simulink model "LLC_Phase_Shift_R2016a"  (R2016a)
settings: Solver=VariableStepAuto  SolverMode=SingleTasking  StartTime=0.0  StopTime=1  RelTol=1e-3
libraries: powerlib x35, simulink x1
settings Model: Creator=20695  LastModifiedBy=20695
settings DataIOCC: ReturnWorkspaceOutputs=on
settings DebuggingCC: UnconnectedInputMsg=none  UnconnectedOutputMsg=none  UnconnectedLineMsg=none  SFUnexpectedBacktrackingDiag=error  SFNoUnconditionalDefaultTransitionDiag=error
settings ModelReferenceCC: EnableRefExpFcnMdlSchedulingChecks=off
settings SFSimCC: SimUseLocalCustomCode=on
settings RTWCC: Description=Generic Real-Time Target  RTWUseLocalCustomCode=on
settings GRTTargetCC: TargetLangStandard=C99 (ISO)
settings ConfigComp: CovMetricSettings=dwe  CovSaveCumulativeToWorkspaceVar=off  CovSaveSingleToWorkspaceVar=off  CovExternalEMLEnable=on

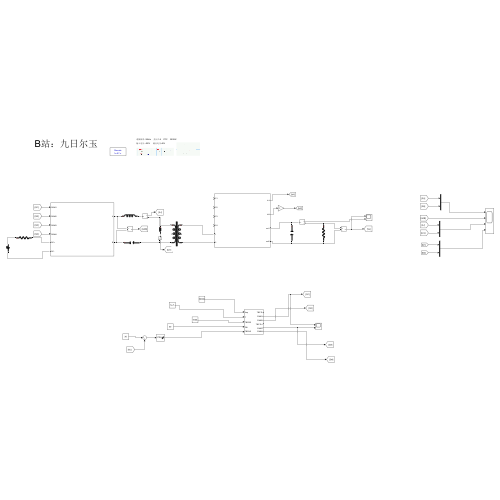
[thumbnail: Simulink's stored preview of the top-level diagram]
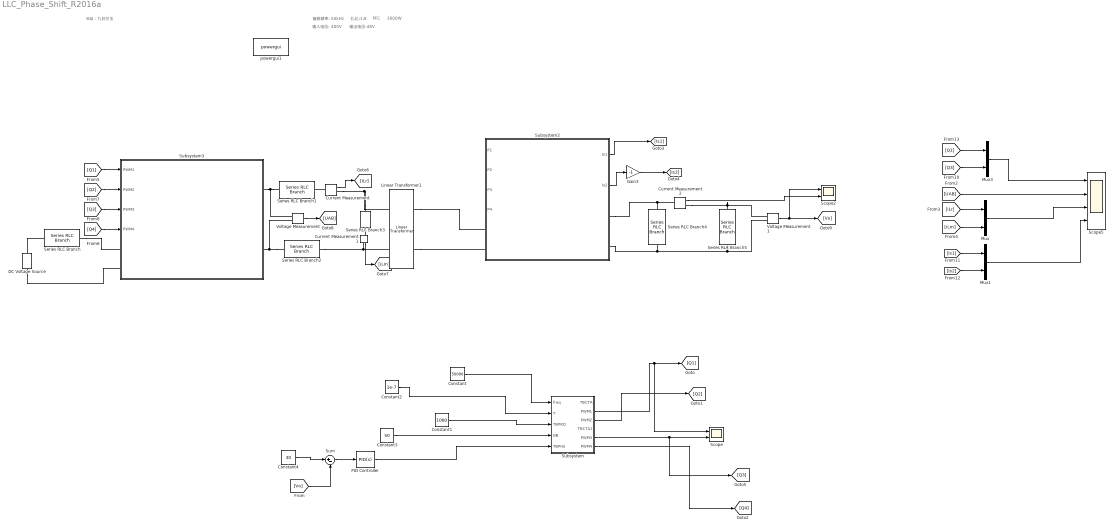
== system LLC_Phase_Shift_R2016a ==
  note: 谐振频率: 50kHz
  note: 输出电压:48V
  note: 3000W
  note: 输入电压: 400V
  note: 扎比:1:8
  note: B站：九日尔玉
  note: PFC
  Constant : Constant  Value=50000
  Constant1 : Constant  Value=1000
  Constant2 : Constant  Value=1e-7
  Constant3 : Constant  Value=50
  Constant4 : Constant  Value=30
  Current Measurement : powerlib/Measurements/Current Measurement  PhasorSimulation=off  OutputType=Complex  PSBequivalent=0
  Current Measurement1 : powerlib/Measurements/Current Measurement  PhasorSimulation=off  OutputType=Complex  PSBequivalent=0
  Current Measurement2 : powerlib/Measurements/Current Measurement  PhasorSimulation=off  OutputType=Complex  PSBequivalent=0
  DC Voltage Source : powerlib/Electrical Sources/DC Voltage Source  Amplitude=400  Measurements=None
  Gain3 : Gain  Gain=-1
  Linear Transformer1 : powerlib/Elements/Linear Transformer  UNITS=SI  NominalPower=[ 3e3 50e3 ]  winding1=[8 0 0]  winding2=[1 0 0]  ThreeWindings=off  winding3=[41.5 1e-4 1e-7]  RmLm=[1e8 0]  Measurements=None  DataType=on
  Mux : Mux  Inputs=2
  Mux1 : Mux  Inputs=2
  Mux3 : Mux  Inputs=2
  PID Controller : simulink/Continuous/PID Controller  Controller=PID  Form=Parallel  TimeDomain=Continuous-time  SampleTime=-1  IntegratorMethod=Forward Euler  ControllerParametersSource=internal  P=100  I=1000  D=0  N=100  UseFilter=on  InitialConditionSource=internal  InitialConditionForIntegrator=0  InitialConditionForFilter=0  DifferentiatorICPrevScaledInput=0  ExternalReset=none  TrackingMode=off  Kt=1  LimitOutput=on  UpperSaturationLimit=1000  LowerSaturationLimit=0  LinearizeAsGain=on  AntiWindupMode=none  Kb=1  POutMin=[]  POutMax=[]  IOutMin=[]  IOutMax=[]  DOutMin=[]  DOutMax=[]  NOutMin=[]  NOutMax=[]  SumOutMin=[]  SumOutMax=[]  SaturationOutMin=[]  SaturationOutMax=[]  PParamMin=[]  PParamMax=[]  IParamMin=[]  IParamMax=[]  DParamMin=[]  DParamMax=[]  NParamMin=[]  NParamMax=[]  KbParamMin=[]  KbParamMax=[]  KtParamMin=[]  KtParamMax=[]  KbOutMin=[]  KbOutMax=[]  KtOutMin=[]  KtOutMax=[]  IntegratorOutMin=[]  IntegratorOutMax=[]  FilterOutMin=[]  FilterOutMax=[]  SumI1OutMin=[]  SumI1OutMax=[]  SumI2OutMin=[]  SumI2OutMax=[]  SumI3OutMin=[]  SumI3OutMax=[]  SumDOutMin=[]  SumDOutMax=[]  DifferentiatorOutMin=[]  DifferentiatorOutMax=[]  IntegratorContinuousStateAttributes=''  IntegratorStateMustResolveToSignalObject=off  IntegratorRTWStateStorageClass=Auto  FilterContinuousStateAttributes=''  FilterStateMustResolveToSignalObject=off  FilterRTWStateStorageClass=Auto
  Scope : Scope  NumInputPorts=2
  Scope2 : Scope  NumInputPorts=2
  Scope5 : Scope  NumInputPorts=4
  Series RLC Branch : powerlib/Elements/Series RLC Branch  LConnTagsString=__new0  RConnTagsString=__new0  BranchType=R  Resistance=0.0001  Inductance=1e-3  SetiL0=off  InitialCurrent=0  Capacitance=1e-6  Setx0=off  InitialVoltage=0  Measurements=None
  Series RLC Branch1 : powerlib/Elements/Series RLC Branch  LConnTagsString=__new0  RConnTagsString=__new0  BranchType=L  Resistance=0.0001  Inductance=0.078e-3  SetiL0=off  InitialCurrent=0  Capacitance=1e-6  Setx0=off  InitialVoltage=0  Measurements=None
  Series RLC Branch2 : powerlib/Elements/Series RLC Branch  LConnTagsString=__new0  RConnTagsString=__new0  BranchType=C  Resistance=0.0001  Inductance=1e-3  SetiL0=off  InitialCurrent=0  Capacitance=130.508e-9  Setx0=off  InitialVoltage=0  Measurements=None
  Series RLC Branch3 : powerlib/Elements/Series RLC Branch  LConnTagsString=__new0  RConnTagsString=__new0  BranchType=L  Resistance=0.0001  Inductance=0.233e-3  SetiL0=off  InitialCurrent=0  Capacitance=1e-6  Setx0=off  InitialVoltage=0  Measurements=None
  Series RLC Branch4 : powerlib/Elements/Series RLC Branch  LConnTagsString=__new0  RConnTagsString=__new0  BranchType=C  Resistance=1  Inductance=1e-3  SetiL0=off  InitialCurrent=0  Capacitance=2e-3  Setx0=on  InitialVoltage=0  Measurements=None
  Series RLC Branch5 : powerlib/Elements/Series RLC Branch  LConnTagsString=__new0  RConnTagsString=__new0  BranchType=R  Resistance=1  Inductance=1e-3  SetiL0=off  InitialCurrent=0  Capacitance=2e-3  Setx0=off  InitialVoltage=0  Measurements=None
  Subsystem : Subsystem
  Subsystem2 : Subsystem  mask{C=0}
  Subsystem3 : Subsystem  mask{C=330e-12}
      mask prompts: C "寄生电容大小"
  Sum : Sum  Inputs=|+-
  Voltage Measurement : powerlib/Measurements/Voltage Measurement  PhasorSimulation=off  OutputType=Complex  PSBequivalent=0
  Voltage Measurement1 : powerlib/Measurements/Voltage Measurement  PhasorSimulation=off  OutputType=Complex  PSBequivalent=0
  powergui1 : powerlib/powergui  Priority=1  SimulationMode=Discrete  SampleTime=1e-7  frequency=60  Iterations=50  frequencyindice=0  Pbase=100e6  ErrMax=1e-4  UnitsV=kV  UnitsW=MW  buscounter=0  FunctionMessages=off  echomessages=off  EnableUseOfTLC=off  CurrentSourceSwitches=off  DisableSnubberDevices=off  DisableRonSwitches=off  DisableVfSwitches=off  DisplayEquations=off  AutomaticDiscreteSolvers=off  SolverType=Tustin/Backward Euler (TBE)  Interpol=off  ExternalGateDelay=off  methode=off  Ts=100  x0status=blocks  SPID=on  SwTol=0  HookPort=off  NonlinearTolerance=1e-4  nMaxIteration=100  ContinueOnMaxIteration=off  RestoreLinks=warning  ResistiveCurrentMeasurement=off  Frange=[0:2:500]  Ylog=off  Xlog=on  ShowGrid=off  save=off  variable=ZData  structure=0  ZoomFFT=off  StartTime=0.0  cycles=1  DisplayStyle=1  fundamental=60  FreqAxis=off  MaxFrequency=1000  frequencyindicesteady=1  RmsSteady=1  display=off
  wires:
  [Q4] -> Subsystem3/4(PWM4)
  [Q2] -> Subsystem3/2(PWM2)
  [Q3] -> Subsystem3/3(PWM3)
  Subsystem2/1(Is1) -> [Is1]
  Current Measurement2/1 -> Scope2/2
  Subsystem2/2(Is2) -> Gain3/1
  Voltage Measurement/1 -> [UAB]
  Voltage Measurement1/1 -> [Vo], Scope2/1
  Gain3/1 -> [Is2]
  [Q1] -> Subsystem3/1(PWM1)
  [UAB] -> Scope5/2
  Mux3/1 -> Scope5/1
  [iLm] -> Mux/2
  Current Measurement/1 -> [iLr]
  [Q3] -> Mux3/2
  Mux/1 -> Scope5/3
  [Q1] -> Mux3/1
  [Is2] -> Mux1/2
  Current Measurement1/1 -> [iLm]
  Mux1/1 -> Scope5/4
  [iLr] -> Mux/1
  [Is1] -> Mux1/1
  Subsystem/2(PWM1) -> Scope/1, [Q1]
  Subsystem/5(PWM3) -> [Q3], Scope/2
  Constant/1 -> Subsystem/1(freq)
  Constant2/1 -> Subsystem/2(T)
  Constant1/1 -> Subsystem/3(TBPRD)
  Constant3/1 -> Subsystem/4(DB)
  PID Controller/1 -> Subsystem/5(TBPHS)
  Subsystem/3(PWM2) -> [Q2]
  Subsystem/6(PWM4) -> [Q4]
  [Vo] -> Sum/2
  Constant4/1 -> Sum/1
  Sum/1 -> PID Controller/1
  connections:
  Series RLC Branch2/LConn1 -- Subsystem3/RConn2 -- Voltage Measurement/LConn2
  Series RLC Branch4/LConn1 -- Subsystem2/RConn1 -- Current Measurement2/LConn1
  Series RLC Branch4/RConn1 -- Subsystem2/RConn2 -- Voltage Measurement1/LConn2 -- Series RLC Branch5/RConn1
  Series RLC Branch3/LConn1 -- Current Measurement/RConn1 -- Linear Transformer1/LConn1
  Series RLC Branch1/LConn1 -- Subsystem3/RConn1 -- Voltage Measurement/LConn1
  Series RLC Branch5/LConn1 -- Current Measurement2/RConn1 -- Voltage Measurement1/LConn1
  Current Measurement1/RConn1 -- Series RLC Branch2/RConn1 -- Linear Transformer1/LConn2
  Linear Transformer1/RConn1 -- Subsystem2/LConn1
  DC Voltage Source/RConn1 -- Series RLC Branch/LConn1
  Current Measurement1/LConn1 -- Series RLC Branch3/RConn1
  Current Measurement/LConn1 -- Series RLC Branch1/RConn1
  Linear Transformer1/RConn2 -- Subsystem2/LConn2
  Series RLC Branch/RConn1 -- Subsystem3/LConn1
  DC Voltage Source/LConn1 -- Subsystem3/LConn2

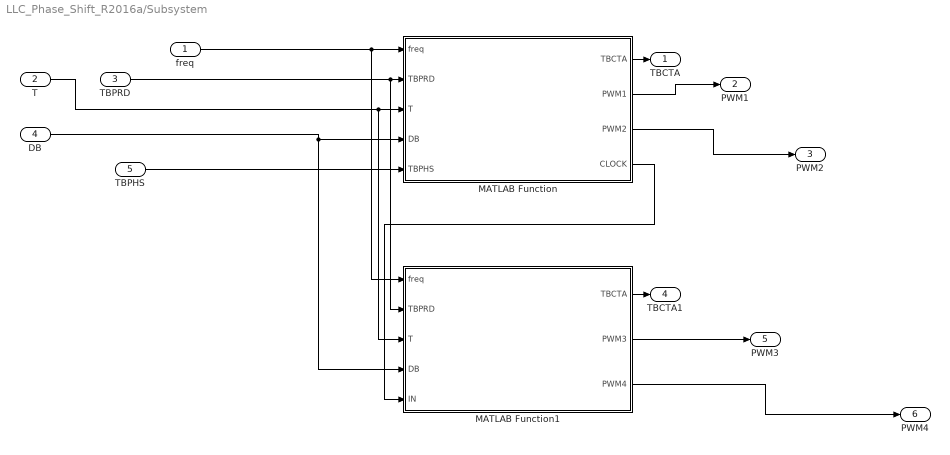
== system LLC_Phase_Shift_R2016a/Subsystem ==
  freq : Inport
  T : Inport  Port=2
  TBPRD : Inport  Port=3
  DB : Inport  Port=4
  TBPHS : Inport  Port=5
  MATLAB Function : MATLAB Function  TreatAsAtomicUnit=on  SystemSampleTime=1e-7
  MATLAB Function1 : MATLAB Function  TreatAsAtomicUnit=on  SystemSampleTime=1e-7
  TBCTA : Outport
  PWM1 : Outport  Port=2
  PWM2 : Outport  Port=3
  TBCTA1 : Outport  Port=4
  PWM3 : Outport  Port=5
  PWM4 : Outport  Port=6
  wires:
  MATLAB Function1/3(PWM4) -> PWM4/1
  freq/1 -> MATLAB Function1/1(freq), MATLAB Function/1(freq)
  MATLAB Function/4(CLOCK) -> MATLAB Function1/5(IN)
  TBPRD/1 -> MATLAB Function1/2(TBPRD), MATLAB Function/2(TBPRD)
  T/1 -> MATLAB Function1/3(T), MATLAB Function/3(T)
  MATLAB Function/1(TBCTA) -> TBCTA/1
  DB/1 -> MATLAB Function1/4(DB), MATLAB Function/4(DB)
  MATLAB Function1/2(PWM3) -> PWM3/1
  TBPHS/1 -> MATLAB Function/5(TBPHS)
  MATLAB Function1/1(TBCTA) -> TBCTA1/1
  MATLAB Function/3(PWM2) -> PWM2/1
  MATLAB Function/2(PWM1) -> PWM1/1

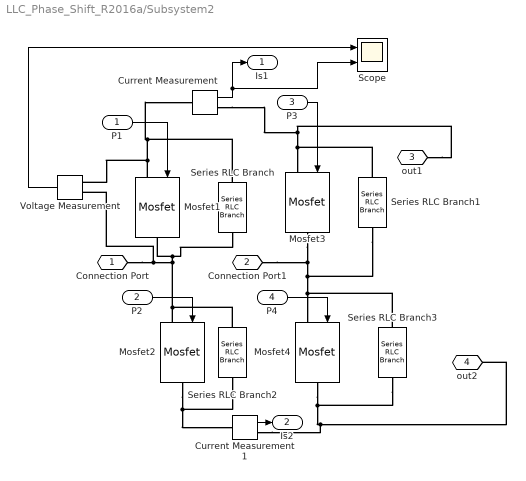
== system LLC_Phase_Shift_R2016a/Subsystem2 ==
  P1 : Inport
  P2 : Inport  Port=2
  P3 : Inport  Port=3
  P4 : Inport  Port=4
  Current Measurement : powerlib/Measurements/Current Measurement  PhasorSimulation=off  OutputType=Complex  PSBequivalent=0
  Current Measurement1 : powerlib/Measurements/Current Measurement  PhasorSimulation=off  OutputType=Complex  PSBequivalent=0
  Mosfet{1..4} (4 alike) : powerlib/Power Electronics/Mosfet  Ron=0.1  Lon=0  Rd=0.01  Vfd=1.5  IC=0  Rs=1e5  Cs=inf  Measurements=off
  Scope : Scope  NumInputPorts=2
  Series RLC Branch{,1..3} (4 alike) : powerlib/Elements/Series RLC Branch  LConnTagsString=__new0  RConnTagsString=__new0  BranchType=C  Resistance=1  Inductance=1e-3  SetiL0=off  InitialCurrent=0  Capacitance=C  Setx0=off  InitialVoltage=0  Measurements=None
  Voltage Measurement : powerlib/Measurements/Voltage Measurement  PhasorSimulation=off  OutputType=Complex  PSBequivalent=0
  Connection Port : PMIOPort  Side=Left
  Connection Port1 : PMIOPort  Port=2  Side=Left
  out1 : PMIOPort  Port=3  Side=Right
  out2 : PMIOPort  Port=4  Side=Right
  Is1 : Outport
  Is2 : Outport  Port=2
  wires:
  P1/1 -> Mosfet1/1
  P2/1 -> Mosfet2/1
  P3/1 -> Mosfet3/1
  P4/1 -> Mosfet4/1
  Current Measurement/1 -> Is1/1, Scope/2
  Current Measurement1/1 -> Is2/1
  Voltage Measurement/1 -> Scope/1
  connections:
  Series RLC Branch2/LConn1 -- Mosfet2/LConn1 -- Voltage Measurement/LConn2 -- Connection Port/RConn1 -- Series RLC Branch/RConn1 -- Mosfet1/RConn1
  Mosfet3/RConn1 -- Connection Port1/RConn1 -- Series RLC Branch1/RConn1 -- Series RLC Branch3/LConn1 -- Mosfet4/LConn1
  out1/RConn1 -- Current Measurement/RConn1 -- Series RLC Branch1/LConn1 -- Mosfet3/LConn1
  out2/RConn1 -- Series RLC Branch3/RConn1 -- Mosfet4/RConn1 -- Current Measurement1/RConn1
  Mosfet1/LConn1 -- Voltage Measurement/LConn1 -- Current Measurement/LConn1 -- Series RLC Branch/LConn1
  Mosfet2/RConn1 -- Series RLC Branch2/RConn1 -- Current Measurement1/LConn1

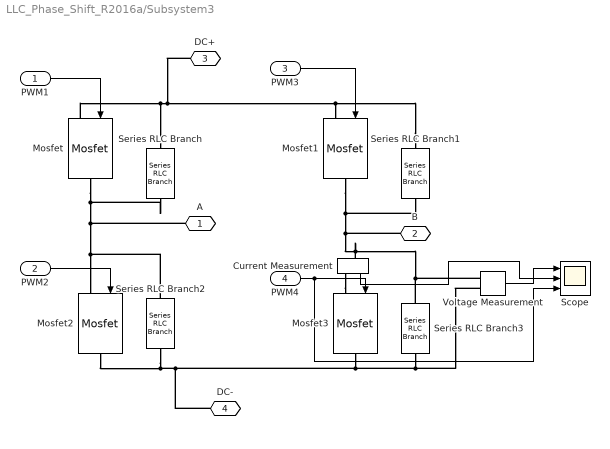
== system LLC_Phase_Shift_R2016a/Subsystem3 ==
  PWM1 : Inport
  PWM2 : Inport  Port=2
  PWM3 : Inport  Port=3
  PWM4 : Inport  Port=4
  Current Measurement : powerlib/Measurements/Current Measurement  PhasorSimulation=off  OutputType=Complex  PSBequivalent=0
  Mosfet{,1..3} (4 alike) : powerlib/Power Electronics/Mosfet  Ron=0.1  Lon=0  Rd=0.01  Vfd=0  IC=0  Rs=1e5  Cs=inf  Measurements=off
  Scope : Scope  NumInputPorts=3
  Series RLC Branch{,1..3} (4 alike) : powerlib/Elements/Series RLC Branch  LConnTagsString=__new0  RConnTagsString=__new0  BranchType=C  Resistance=1  Inductance=1e-3  SetiL0=off  InitialCurrent=0  Capacitance=C  Setx0=off  InitialVoltage=0  Measurements=None
  Voltage Measurement : powerlib/Measurements/Voltage Measurement  PhasorSimulation=off  OutputType=Complex  PSBequivalent=0
  A : PMIOPort  Side=Right
  B : PMIOPort  Port=2  Side=Right
  DC+ : PMIOPort  Port=3  Side=Left
  DC- : PMIOPort  Port=4  Side=Left
  wires:
  PWM1/1 -> Mosfet/1
  PWM4/1 -> Scope/3, Mosfet3/1
  PWM3/1 -> Mosfet1/1
  PWM2/1 -> Mosfet2/1
  Current Measurement/1 -> Scope/2
  Voltage Measurement/1 -> Scope/1
  connections:
  Series RLC Branch3/LConn1 -- Series RLC Branch1/RConn1 -- Mosfet1/RConn1 -- B/RConn1 -- Current Measurement/LConn1 -- Voltage Measurement/LConn1
  Series RLC Branch1/LConn1 -- Mosfet1/LConn1 -- Mosfet/LConn1 -- Series RLC Branch/LConn1 -- DC+/RConn1
  Series RLC Branch/RConn1 -- Mosfet/RConn1 -- Series RLC Branch2/LConn1 -- Mosfet2/LConn1 -- A/RConn1
  Mosfet2/RConn1 -- Series RLC Branch2/RConn1 -- Voltage Measurement/LConn2 -- Series RLC Branch3/RConn1 -- Mosfet3/RConn1 -- DC-/RConn1
  Current Measurement/RConn1 -- Mosfet3/LConn1

== matlab function LLC_Phase_Shift_R2016a/Subsystem/MATLAB Function1 ==
  data: freq input; TBCTA output; TBPRD input; T input; DB input; PWM3 output; PWM4 output; IN input
function [TBCTA,PWM3,PWM4]  = fcn(freq,TBPRD,T,DB,IN)
persistent out1;
if isempty(out1)
    out1=0;
end
persistent flag;
if isempty(flag)
    flag=0;
end

persistent P1;
if isempty(P1)
    P1=0;
end
persistent P2;
if isempty(P2)
    P2=0;
end


if IN == 1
    out1 = 0;
end
Ts = 1/freq;
if flag == 0
    out1 = out1 + TBPRD/(Ts/2/T);%增计算
    if out1 > TBPRD-DB
        P1 = 0;
    end

else
    out1 = out1 -  TBPRD/(Ts/2/T);%减计算
    if out1 < DB
        P2 = 0;
    end
end
if out1 > TBPRD
   out1 = TBPRD;
   flag = 1;
   P1 = 0;
   P2 = 1;
end
if out1 < 0
   out1 = 0;
   flag = 0;
   P1 = 1;
   P2 = 0;
end

PWM3 = P1;
PWM4 = P2;

TBCTA = out1;

== matlab function LLC_Phase_Shift_R2016a/Subsystem/MATLAB Function ==
  data: freq input; TBCTA output; TBPRD input; T input; DB input; PWM1 output; PWM2 output; CLOCK output; TBPHS input
function [TBCTA,PWM1,PWM2,CLOCK]  = fcn(freq,TBPRD,T,DB,TBPHS)
persistent out1;
if isempty(out1)
    out1=0;
end
persistent flag;
if isempty(flag)
    flag=0;
end

persistent P1;
if isempty(P1)
    P1=0;
end
persistent P2;
if isempty(P2)
    P2=0;
end
persistent flag1;
if isempty(flag1)
    flag1=0;
end
CLOCK = 0;

Ts = 1/freq;
if flag == 0
    out1 = out1 + TBPRD/(Ts/2/T);%增计算
    if out1 > TBPRD-DB
        P1 = 0;
    end

    if out1>=TBPHS-TBPRD/(Ts/2/T)&&flag1 == 1
        CLOCK = 1;
        flag1 = 0;
    end
else
    out1 = out1 -  TBPRD/(Ts/2/T);%减计算
    if out1 < DB
        P2 = 0;
    end
    flag1 = 1;
end
if out1 > TBPRD
   out1 = TBPRD;
   flag = 1;
   P1 = 0;
   P2 = 1;
end
if out1 < 0
   out1 = 0;
   flag = 0;
   P1 = 1;
   P2 = 0;
end
PWM1 = P1;
PWM2 = P2;
TBCTA = out1;
